simulink library "focLib"  (R2023a)
settings: Solver=VariableStepAuto  StartTime=0.0  StopTime=10.0  RelTol=1e-3
undefined symbols (not defined in the file): availableSpeedModes, ctrl_limits, Down, focp_tune_cur_Ki, focp_tune_cur_Kp, focp_tune_iq_max, focp_tune_iq_min, focp_tune_spd_Ki, focp_tune_spd_Kp, focp_tune_udc_max, GPTRIP1SEL, inverter_DRV8300, PI_params, pmsm_ECI6360, PU_System, target_f2838, Ts, Ts_motor, Ts_simulink, Ts_speed, TZ1, Up
libraries: simulink x31, c2802xlib x12, idelinklib_common x8, mcbcontrolslib x8, c280xlib x7, mcbpositiondecoderlib x7, slpidlib x5, c2837xDlib x2, c2838xlib x1, autolibpmsminterior x1, mcbplantlib x1, autolibpmsmexterior x1
(part 2 of 3)

== system focLib/Speed Control/Speed calculator ==
  Speed_Ref_PU : Inport
  speedMode : Inport  Port=2
  Gain : Gain  Gain=floor(PU_System.N_base/availableSpeedModes)  OutDataTypeStr=fixdt(1,32,17)  RndMeth=Ceiling
  Product : Product  OutDataTypeStr=fixdt(1,32,17)
  Subsystem : Subsystem  Commented=through
  rpm2PU : Gain  Gain=1/PU_System.N_base  OutMax=1  OutDataTypeStr=fixdt(1,32,17)
  N_Ref : Outport
  wires:
  Subsystem/1(Out1) -> N_Ref/1
  rpm2PU/1 -> Subsystem/1(In1)
  Product/1 -> rpm2PU/1
  speedMode/1 -> Product/1
  Gain/1 -> Product/2
  Speed_Ref_PU/1 -> Gain/1

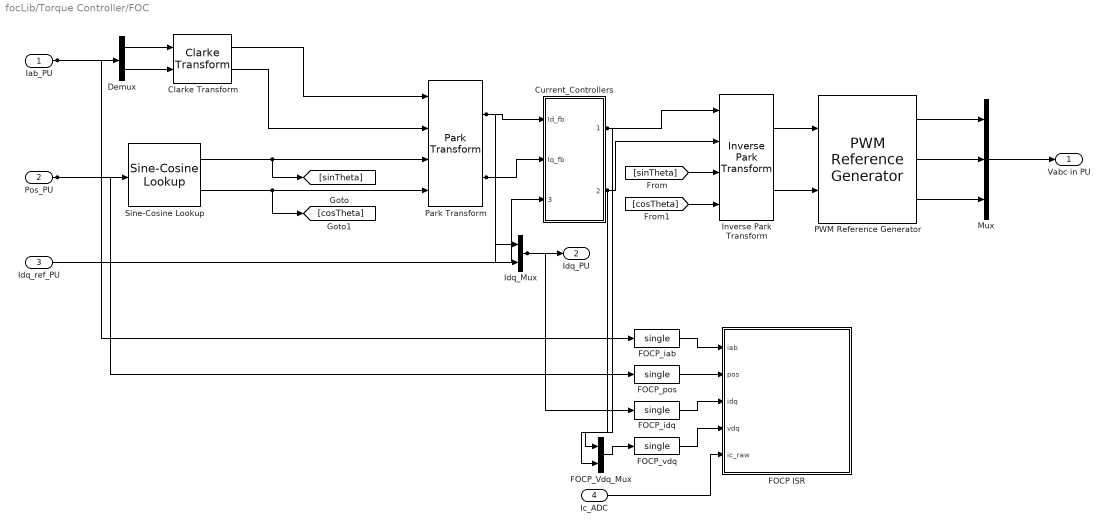
== system focLib/Torque Controller/FOC ==
  Iab_PU : Inport
  Pos_PU : Inport  Port=2
  Idq_ref_PU : Inport  Port=3
  Ic_ADC : Inport  Port=4
  Clarke Transform : mcbcontrolslib/Clarke Transform  VariantControl=Variant2
      settings: LibrarySourceBlock=mcbhdllib/Controls/Math Transforms/Clarke Transform
  Current_Controllers : Subsystem
  Demux : Demux  Outputs=2
  FOCP ISR : MATLAB Function  TreatAsAtomicUnit=on
  FOCP_Vdq_Mux : Mux  Inputs=2
  FOCP_iab : DataTypeConversion  OutDataTypeStr=single  SaturateOnIntegerOverflow=off  RndMeth=Floor
  FOCP_idq : DataTypeConversion  OutDataTypeStr=single  SaturateOnIntegerOverflow=off  RndMeth=Floor
  FOCP_pos : DataTypeConversion  OutDataTypeStr=single  SaturateOnIntegerOverflow=off  RndMeth=Floor
  FOCP_vdq : DataTypeConversion  OutDataTypeStr=single  SaturateOnIntegerOverflow=off  RndMeth=Floor
  Idq_Mux : Mux  Inputs=2
  Inverse Park Transform : mcbcontrolslib/Inverse Park Transform  AxisAlignment=D-axis
      settings: LibrarySourceBlock=mcbhdllib/Controls/Math Transforms/Inverse Park Transform
  Mux : Mux  Inputs=3
  PWM Reference Generator : mcbcontrolslib/PWM Reference Generator  inSignal=Valphabeta  modType=SVM: space vector modulation
      settings: LibrarySourceBlock=mcblib/Controls/Math Transforms/PWM Reference Generator
  Park Transform : mcbcontrolslib/Park Transform  AxisAlignment=D-axis
      settings: LibrarySourceBlock=mcbhdllib/Controls/Math Transforms/Park Transform
  Sine-Cosine Lookup : mcbcontrolslib/Sine-Cosine Lookup  AngleInput=Per-unit  N_points=1024
      settings: LibrarySourceBlock=mcblib/Controls/Math Transforms/Sine-Cosine Lookup
  Vabc in PU : Outport
  Idq_PU : Outport  Port=2
  wires:
  Current_Controllers/2(Vq_ref) -> Inverse Park Transform/2, FOCP_Vdq_Mux/2
  Current_Controllers/1(Vd_ref) -> Inverse Park Transform/1, FOCP_Vdq_Mux/1
  Pos_PU/1 -> Sine-Cosine Lookup/1, FOCP_pos/1
  Mux/1 -> Vabc in PU/1
  PWM Reference Generator/3 -> Mux/3
  PWM Reference Generator/2 -> Mux/2
  PWM Reference Generator/1 -> Mux/1
  Inverse Park Transform/2 -> PWM Reference Generator/2
  Inverse Park Transform/1 -> PWM Reference Generator/1
  [cosTheta] -> Inverse Park Transform/4
  [sinTheta] -> Inverse Park Transform/3
  Idq_ref_PU/1 -> Current_Controllers/3(Idq_ref_PU)
  Park Transform/2 -> Current_Controllers/2(Iq_fb), Idq_Mux/2
  Park Transform/1 -> Current_Controllers/1(Id_fb), Idq_Mux/1
  Sine-Cosine Lookup/2 -> Park Transform/4, [cosTheta]
  Sine-Cosine Lookup/1 -> Park Transform/3, [sinTheta]
  Clarke Transform/2 -> Park Transform/2
  Clarke Transform/1 -> Park Transform/1
  Demux/2 -> Clarke Transform/2
  Demux/1 -> Clarke Transform/1
  Iab_PU/1 -> Demux/1, FOCP_iab/1
  Idq_Mux/1 -> Idq_PU/1, FOCP_idq/1
  FOCP_iab/1 -> FOCP ISR/1(iab)
  FOCP_pos/1 -> FOCP ISR/2(pos)
  FOCP_idq/1 -> FOCP ISR/3(idq)
  FOCP_vdq/1 -> FOCP ISR/4(vdq)
  FOCP_Vdq_Mux/1 -> FOCP_vdq/1
  Ic_ADC/1 -> FOCP ISR/5(ic_raw)

== system focLib/Torque Controller/Iab_Meas_ADC ==
  ADC : c2802xlib/ADC  blkParamProc=C2000_Type4  ADCModule=B  samplingMode=Single sample mode  ADCResolution=12-bit (Single-ended input)  useSOC1=SOC0  useSOC2=SOC0_SOC1  SOCAcquisitionWindow=60  SOCTriggerSource=ePWM6_ADCSOCA  SOCInterruptTrigger=No ADCINT  Ts=-1  dType=uint16  postInterrupt=off  interruptSel=ADCINT1  ADCINTContinuous=on  endma=off  chdma=1  conv1=ADCINA0  conv2=ADCINA0 and ADCINB0  conv1_Type4=ADCIN0  conv2_Type4=ADCIN0 and ADCIN1
      settings: LibrarySourceBlock=c2838xlib/ADC
  ADC1 : c2802xlib/ADC  blkParamProc=C2000_Type4  ADCModule=B  samplingMode=Single sample mode  ADCResolution=12-bit (Single-ended input)  useSOC1=SOC1  useSOC2=SOC0_SOC1  SOCAcquisitionWindow=60  SOCTriggerSource=ePWM6_ADCSOCA  SOCInterruptTrigger=No ADCINT  Ts=-1  dType=uint16  postInterrupt=on  interruptSel=ADCINT1  ADCINTContinuous=on  endma=off  chdma=1  conv1=ADCINA0  conv2=ADCINA0 and ADCINB0  conv1_Type4=ADCIN2  conv2_Type4=ADCIN0 and ADCIN1
      settings: LibrarySourceBlock=c2838xlib/ADC
  ADC_IC : c2802xlib/ADC  blkParamProc=C2000_Type4  ADCModule=B  samplingMode=Single sample mode  ADCResolution=12-bit (Single-ended input)  useSOC1=SOC4  useSOC2=SOC0_SOC1  SOCAcquisitionWindow=60  SOCTriggerSource=ePWM6_ADCSOCA  SOCInterruptTrigger=No ADCINT  Ts=-1  dType=uint16  postInterrupt=off  interruptSel=ADCINT1  ADCINTContinuous=on  endma=off  chdma=1  conv1=ADCINA0  conv2=ADCINA0 and ADCINB0  conv1_Type4=ADCIN3  conv2_Type4=ADCIN0 and ADCIN1
      settings: LibrarySourceBlock=c2838xlib/ADC
  Mux : Mux  Inputs=2
  Iab_ADC : Outport
  Ic_ADC : Outport  Port=2
  wires:
  ADC1/1 -> Mux/2
  ADC/1 -> Mux/1
  Mux/1 -> Iab_ADC/1
  ADC_IC/1 -> Ic_ADC/1

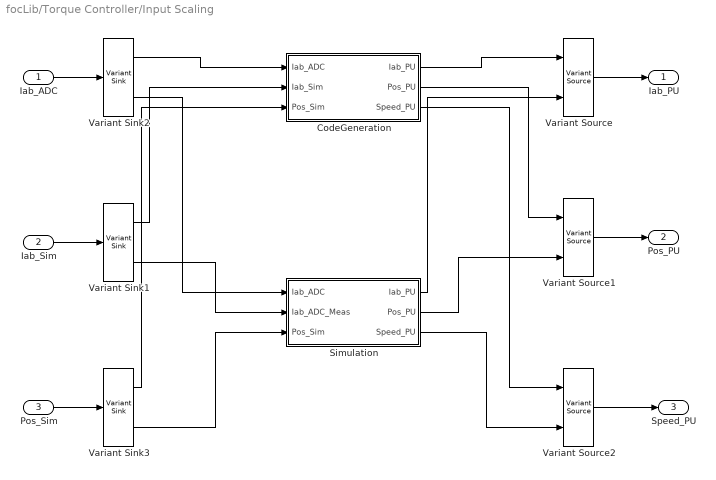
== system focLib/Torque Controller/Input Scaling ==
  Iab_ADC : Inport
  Iab_Sim : Inport  Port=2
  Pos_Sim : Inport  Port=3
  CodeGeneration : Subsystem
  Simulation : Subsystem
  Variant Sink1 : VariantSink  VariantControlMode=sim codegen switching
  Variant Sink2 : VariantSink  VariantControlMode=sim codegen switching
  Variant Sink3 : VariantSink  VariantControlMode=sim codegen switching
  Variant Source : VariantSource  VariantControlMode=sim codegen switching
  Variant Source1 : VariantSource  VariantControlMode=sim codegen switching
  Variant Source2 : VariantSource  VariantControlMode=sim codegen switching
  Iab_PU : Outport
  Pos_PU : Outport  Port=2
  Speed_PU : Outport  Port=3
  wires:
  Variant Source2/1 -> Speed_PU/1
  Variant Source1/1 -> Pos_PU/1
  Variant Source/1 -> Iab_PU/1
  CodeGeneration/3(Speed_PU) -> Variant Source2/1
  Simulation/3(Speed_PU) -> Variant Source2/2
  Simulation/2(Pos_PU) -> Variant Source1/2
  CodeGeneration/2(Pos_PU) -> Variant Source1/1
  Simulation/1(Iab_PU) -> Variant Source/2
  CodeGeneration/1(Iab_PU) -> Variant Source/1
  Variant Sink3/2 -> Simulation/3(Pos_Sim)
  Variant Sink1/2 -> Simulation/2(Iab_ADC_Meas)
  Variant Sink2/2 -> Simulation/1(Iab_ADC)
  Variant Sink3/1 -> CodeGeneration/3(Pos_Sim)
  Variant Sink1/1 -> CodeGeneration/2(Iab_Sim)
  Variant Sink2/1 -> CodeGeneration/1(Iab_ADC)
  Iab_ADC/1 -> Variant Sink2/1
  Iab_Sim/1 -> Variant Sink1/1
  Pos_Sim/1 -> Variant Sink3/1

== system focLib/Torque Controller/Output ==
  Scaled_DC : Inport
  CodeGeneration : Subsystem
  Scope : Scope
  Simulation : Subsystem
  Variant Sink : VariantSink  VariantControlMode=sim codegen switching
  Duty Cycle : Outport
  wires:
  Variant Sink/2 -> Simulation/1(Input)
  Variant Sink/1 -> CodeGeneration/1(In1)
  Simulation/1(Output) -> Duty Cycle/1, Scope/1
  Scaled_DC/1 -> Variant Sink/1

== system focLib/Torque Controller/PWM1 ==
  Scaled_DC_PWM1 : Inport
  Freemode_Sig : Inport  Port=2
  Constant : Constant  Value=0  OutDataTypeStr=fixdt(1,32,17)  SampleTime=-1
  Constant1 : Constant  OutDataTypeStr=fixdt(1,32,17)  SampleTime=-1
  Switch : Switch  Criteria=u2 > Threshold  SaturateOnIntegerOverflow=off  InputSameDT=off  OutDataTypeStr=Inherit: Same as first input
  Switch1 : Switch  Criteria=u2 > Threshold  SaturateOnIntegerOverflow=off  InputSameDT=off  OutDataTypeStr=Inherit: Same as first input
  WA : Outport
  WB : Outport  Port=2
  wires:
  Constant1/1 -> Switch1/1
  Constant/1 -> Switch/1
  Scaled_DC_PWM1/1 -> Switch1/3, Switch/3
  Switch1/1 -> WB/1
  Switch/1 -> WA/1
  Freemode_Sig/1 -> Switch/2, Switch1/2

== system focLib/Torque Controller/PWM2 ==
  Scaled_DC_PWM2 : Inport
  Freemode_Sig : Inport  Port=2
  Constant : Constant  Value=0  OutDataTypeStr=fixdt(1,32,17)  SampleTime=-1
  Constant1 : Constant  OutDataTypeStr=fixdt(1,32,17)  SampleTime=-1
  Switch : Switch  Criteria=u2 > Threshold  SaturateOnIntegerOverflow=off  InputSameDT=off  OutDataTypeStr=Inherit: Same as first input
  Switch1 : Switch  Criteria=u2 > Threshold  SaturateOnIntegerOverflow=off  InputSameDT=off  OutDataTypeStr=Inherit: Same as first input
  WA : Outport
  WB : Outport  Port=2
  wires:
  Scaled_DC_PWM2/1 -> Switch/3, Switch1/3
  Constant1/1 -> Switch1/1
  Freemode_Sig/1 -> Switch1/2, Switch/2
  Constant/1 -> Switch/1
  Switch1/1 -> WB/1
  Switch/1 -> WA/1

== system focLib/Torque Controller/PWM3 ==
  Scaled_DC_PWM3 : Inport
  Freemode_Sig : Inport  Port=2
  Constant : Constant  Value=0  OutDataTypeStr=fixdt(1,32,17)  SampleTime=-1
  Constant1 : Constant  OutDataTypeStr=fixdt(1,32,17)  SampleTime=-1
  Switch : Switch  Criteria=u2 > Threshold  SaturateOnIntegerOverflow=off  InputSameDT=off  OutDataTypeStr=Inherit: Same as first input
  Switch1 : Switch  Criteria=u2 > Threshold  SaturateOnIntegerOverflow=off  InputSameDT=off  OutDataTypeStr=Inherit: Same as first input
  WA : Outport
  WB : Outport  Port=2
  wires:
  Scaled_DC_PWM3/1 -> Switch/3, Switch1/3
  Constant1/1 -> Switch1/1
  Freemode_Sig/1 -> Switch/2, Switch1/2
  Constant/1 -> Switch/1
  Switch1/1 -> WB/1
  Switch/1 -> WA/1

== system focLib/Torque Controller/Scaling DutyCycles ==
  Unscaled_DC : Inport
  CodeGen : Subsystem
  Demux : Demux  Outputs=3
  Sim : Subsystem
  Variant Sink : VariantSink  VariantControlMode=sim codegen switching
  Variant Source : VariantSource  VariantControlMode=sim codegen switching
  Scaled_DC_PWM1 : Outport
  Scaled_DC_PWM2 : Outport  Port=2
  Scaled_DC_PWM3 : Outport  Port=3
  wires:
  CodeGen/1(Out1) -> Variant Source/1
  Variant Sink/1 -> CodeGen/1(In1)
  Variant Sink/2 -> Sim/1(In1)
  Sim/1(Out1) -> Variant Source/2
  Unscaled_DC/1 -> Variant Sink/1
  Variant Source/1 -> Demux/1
  Demux/3 -> Scaled_DC_PWM3/1
  Demux/2 -> Scaled_DC_PWM2/1
  Demux/1 -> Scaled_DC_PWM1/1

== system focLib/ADC Offset Function/Calculate ADC Offset /For Iterator Subsystem ==
  ADC_B_IN0 : c2802xlib/ADC  Priority=20  blkParamProc=C2000_Type4  ADCModule=B  samplingMode=Single sample mode  ADCResolution=12-bit (Single-ended input)  useSOC1=SOC2  useSOC2=SOC0_SOC1  SOCAcquisitionWindow=60  SOCTriggerSource=Software  SOCInterruptTrigger=No ADCINT  Ts=-1  dType=uint16  postInterrupt=off  interruptSel=ADCINT1  ADCINTContinuous=on  endma=off  chdma=1  conv1=ADCINA0  conv2=ADCINA0 and ADCINB0  conv1_Type4=ADCIN0  conv2_Type4=ADCIN0 and ADCIN1
  ADC_B_IN2 : c2802xlib/ADC  Priority=20  blkParamProc=C2000_Type4  ADCModule=B  samplingMode=Single sample mode  ADCResolution=12-bit (Single-ended input)  useSOC1=SOC3  useSOC2=SOC0_SOC1  SOCAcquisitionWindow=60  SOCTriggerSource=Software  SOCInterruptTrigger=No ADCINT  Ts=-1  dType=uint16  postInterrupt=off  interruptSel=ADCINT1  ADCINTContinuous=on  endma=off  chdma=1  conv1=ADCINA0  conv2=ADCINA0 and ADCINB0  conv1_Type4=ADCIN2  conv2_Type4=ADCIN0 and ADCIN1
  For Iterator : ForIterator  IterationLimit=16  IterationVariableDataType=uint16
  If : If  IfExpression=u1 > 8  ShowElse=off
  If Action Subsystem : Subsystem  TreatAsAtomicUnit=on
  Out1 : Outport
  Out2 : Outport  Port=2
  wires:
  If/1 -> If Action Subsystem/Action
  If Action Subsystem/2(Out2) -> Out2/1
  If Action Subsystem/1(Out1) -> Out1/1
  ADC_B_IN2/1 -> If Action Subsystem/2(In2)
  ADC_B_IN0/1 -> If Action Subsystem/1(In1)
  For Iterator/1 -> If/1

== system focLib/ADC Offset Function/Calculate ADC Offset /If Action Subsystem ==
  In1 : Inport
  Action Port : ActionPort
  Data Store Write1 : DataStoreWrite  DataStoreName=IaOffset  IndexOptions=Index vector (dialog)  Indices=1  OutputSizes=1
  wires:
  In1/1 -> Data Store Write1/1

== system focLib/ADC Offset Function/Calculate ADC Offset /If Action Subsystem1 ==
  Action Port : ActionPort
  Constant : Constant  Value=inverter_DRV8300.CtSensAOffset  OutDataTypeStr=Inherit: Inherit via back propagation
  Data Store Write1 : DataStoreWrite  DataStoreName=IaOffset  IndexOptions=Index vector (dialog)  Indices=1  OutputSizes=1
  wires:
  Constant/1 -> Data Store Write1/1

== system focLib/ADC Offset Function/Calculate ADC Offset /If Action Subsystem2 ==
  In1 : Inport
  Action Port : ActionPort
  Data Store Write2 : DataStoreWrite  DataStoreName=IbOffset  IndexOptions=Index vector (dialog)  Indices=1  OutputSizes=1
  wires:
  In1/1 -> Data Store Write2/1

== system focLib/ADC Offset Function/Calculate ADC Offset /If Action Subsystem3 ==
  Action Port : ActionPort
  Constant1 : Constant  Value=inverter_DRV8300.CtSensBOffset  OutDataTypeStr=Inherit: Inherit via back propagation
  Data Store Write2 : DataStoreWrite  DataStoreName=IbOffset  IndexOptions=Index vector (dialog)  Indices=1  OutputSizes=1
  wires:
  Constant1/1 -> Data Store Write2/1

== system focLib/Hall Sensor A/Capture Event Selection/Output 0 ==
  Action Port : ActionPort
  Constant : Constant  Value=0  OutDataTypeStr=boolean  SampleTime=-1
  Out1 : Outport
  wires:
  Constant/1 -> Out1/1

== system focLib/Hall Sensor A/Capture Event Selection/Output 1 ==
  Action Port : ActionPort
  Constant : Constant  OutDataTypeStr=boolean  SampleTime=-1
  Out1 : Outport
  wires:
  Constant/1 -> Out1/1

== system focLib/Hall Sensor B/Capture Event Selection/Output 0 ==
  Action Port : ActionPort
  Constant : Constant  Value=0  OutDataTypeStr=boolean  SampleTime=-1
  Out1 : Outport
  wires:
  Constant/1 -> Out1/1

== system focLib/Hall Sensor B/Capture Event Selection/Output 1 ==
  Action Port : ActionPort
  Constant : Constant  OutDataTypeStr=boolean  SampleTime=-1
  Out1 : Outport
  wires:
  Constant/1 -> Out1/1

== system focLib/Hall Sensor C/Capture Event Selection/Output 0 ==
  Action Port : ActionPort
  Constant : Constant  Value=0  OutDataTypeStr=boolean  SampleTime=-1
  Out1 : Outport
  wires:
  Constant/1 -> Out1/1

== system focLib/Hall Sensor C/Capture Event Selection/Output 1 ==
  Action Port : ActionPort
  Constant : Constant  OutDataTypeStr=boolean  SampleTime=-1
  Out1 : Outport
  wires:
  Constant/1 -> Out1/1

== system focLib/Input Controller/SpeedCommand_CodeGen/Check for SpeedRef ==
  In1 : Inport
  If : If  IfExpression=u1 > 4000
  If Action Subsystem : Subsystem  TreatAsAtomicUnit=on
  If Action Subsystem1 : Subsystem  TreatAsAtomicUnit=on
  Merge : Merge
  Out1 : Outport
  wires:
  If Action Subsystem1/1(Out1) -> Merge/2
  If Action Subsystem/1(Out1) -> Merge/1
  If/2 -> If Action Subsystem1/Action
  If/1 -> If Action Subsystem/Action
  Merge/1 -> Out1/1
  In1/1 -> If/1, If Action Subsystem1/1(In1)

== system focLib/Inverter and Motor - Plant Model/Simulation/Inverter ==
  Duty_abc : Inport
  Average-Value Inverter : mcbplantlib/Average-Value Inverter
  Constant2 : Constant  Value=inverter_DRV8300.V_dc  OutDataTypeStr=single  SampleTime=-1
  Data Type Conversion1 : DataTypeConversion  OutDataTypeStr=single  RndMeth=Simplest  SaturateOnIntegerOverflow=off
  Rate Transition3 : RateTransition  Integrity=off  OutPortSampleTime=Ts_inverter
  Vabc : Outport  VectorParamsAs1DForOutWhenUnconnected=off
  wires:
  Average-Value Inverter/1 -> Vabc/1
  Constant2/1 -> Average-Value Inverter/2
  Rate Transition3/1 -> Average-Value Inverter/1
  Data Type Conversion1/1 -> Rate Transition3/1
  Duty_abc/1 -> Data Type Conversion1/1

== system focLib/Inverter and Motor - Plant Model/Simulation/Load_Profile (Torque) ==
  Data Type Conversion : DataTypeConversion  OutDataTypeStr=single  SaturateOnIntegerOverflow=off  RndMeth=Floor
  IIR Filter : mcbcontrolslib/IIR Filter  VariantControl=Low Pass Filter  VariantSelect=Low-pass  Filter_constant=0.01  advancedSettings=off  Ts=50e-6  cutOff_freq=32.1525
  T_load : Step  Time=5  Before=0.1*pmsm_ECI6360.T_rated  After=0.1*pmsm_ECI6360.T_rated  SampleTime=Ts_simulink
  Load_Trq : Outport  VectorParamsAs1DForOutWhenUnconnected=off
  wires:
  IIR Filter/1 -> Load_Trq/1
  Data Type Conversion/1 -> IIR Filter/1
  T_load/1 -> Data Type Conversion/1

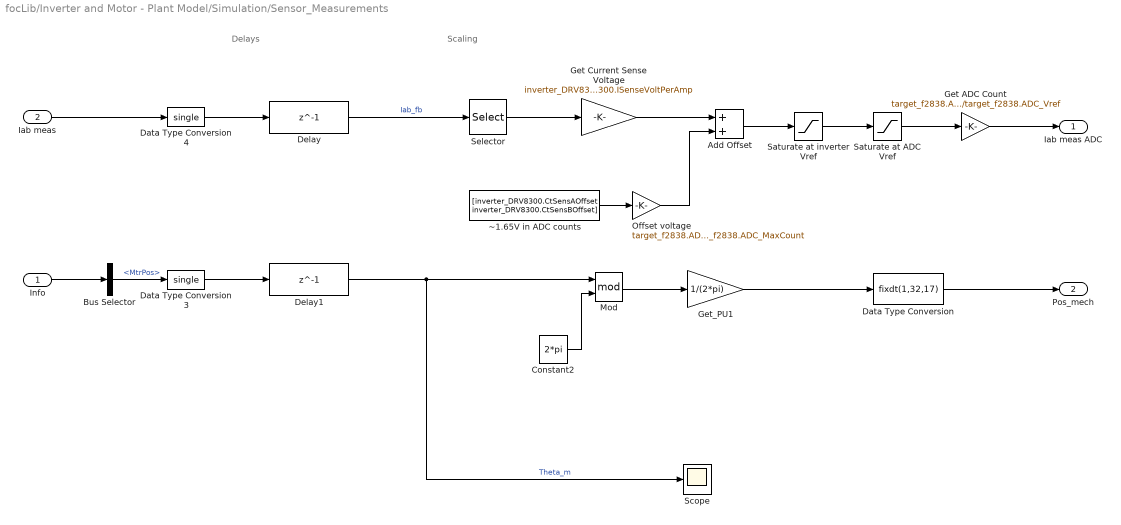
== system focLib/Inverter and Motor - Plant Model/Simulation/Sensor_Measurements ==
  note: Delays
  note: Scaling
  Info : Inport
  Iab meas : Inport  Port=2
  Add Offset : Sum  RndMeth=Simplest
  Bus Selector : BusSelector  OutputSignals=MtrPos
  Constant2 : Constant  Value=2*pi  OutDataTypeStr=single  SampleTime=-1
  Data Type Conversion : DataTypeConversion  OutDataTypeStr=fixdt(1,32,17)  SaturateOnIntegerOverflow=off  RndMeth=Floor
  Data Type Conversion3 : DataTypeConversion  OutDataTypeStr=single  RndMeth=Simplest  SaturateOnIntegerOverflow=off
  Data Type Conversion4 : DataTypeConversion  OutDataTypeStr=single  RndMeth=Simplest  SaturateOnIntegerOverflow=off
  Delay : Delay  DelayLength=1
  Delay1 : Delay  DelayLength=1
  Get ADC Count : Gain  Gain=target_f2838.ADC_MaxCount/target_f2838.ADC_Vref  OutMin=0  OutMax=target_f2838.ADC_MaxCount  OutDataTypeStr=uint16  RndMeth=Simplest
  Get Current Sense Voltage : Gain  Gain=inverter_DRV8300.invertingAmp*inverter_DRV8300.ISenseVoltPerAmp  RndMeth=Simplest  OutDataTypeStr=Inherit: Same as input
  Get_PU1 : Gain  Gain=1/(2*pi)  RndMeth=Simplest  OutDataTypeStr=Inherit: Same as input
  Mod : Math  Operator=mod
  Offset voltage : Gain  Gain=target_f2838.ADC_Vref / target_f2838.ADC_MaxCount  RndMeth=Simplest
  Saturate at ADC Vref : Saturate  UpperLimit=target_f2838.ADC_Vref  LowerLimit=0
  Saturate at inverter Vref : Saturate  UpperLimit=inverter_DRV8300.ISenseVref  LowerLimit=0
  Scope : Scope
  Selector : Selector  InputPortWidth=3  IndexOptions=Index vector (dialog)  Indices=[1 2]  OutputSizes=1
  ~1.65V in ADC counts : Constant  Value=[inverter_DRV8300.CtSensAOffset inverter_DRV8300.CtSensBOffset]  OutDataTypeStr=uint16  SampleTime=-1
  Iab meas ADC : Outport  VectorParamsAs1DForOutWhenUnconnected=off
  Pos_mech : Outport  Port=2
  wires:
  Data Type Conversion/1 -> Pos_mech/1
  Get Current Sense Voltage/1 -> Add Offset/1
  ~1.65V in ADC counts/1 -> Offset voltage/1
  Saturate at ADC Vref/1 -> Get ADC Count/1
  Offset voltage/1 -> Add Offset/2
  Get ADC Count/1 -> Iab meas ADC/1
  Add Offset/1 -> Saturate at inverter Vref/1
  Saturate at inverter Vref/1 -> Saturate at ADC Vref/1
  Selector/1 -> Get Current Sense Voltage/1
  Delay1/1 -> Mod/1, Scope/1  "Theta_m"
  Mod/1 -> Get_PU1/1
  Constant2/1 -> Mod/2
  Bus Selector/1 -> Data Type Conversion3/1  "<MtrPos>"
  Get_PU1/1 -> Data Type Conversion/1
  Data Type Conversion3/1 -> Delay1/1
  Info/1 -> Bus Selector/1
  Iab meas/1 -> Data Type Conversion4/1
  Data Type Conversion4/1 -> Delay/1
  Delay/1 -> Selector/1  "Iab_fb"

== system focLib/Speed Control/Mechanical_Freemode_Check/If Action Subsystem ==
  Action Port : ActionPort
  Constant : Constant  OutDataTypeStr=boolean  SampleTime=-1
  Out1 : Outport
  wires:
  Constant/1 -> Out1/1

== system focLib/Speed Control/Mechanical_Freemode_Check/If Action Subsystem1 ==
  Freemode_Sig_Dig : Inport
  Action Port : ActionPort
  Out1 : Outport
  wires:
  Freemode_Sig_Dig/1 -> Out1/1

== system focLib/Speed Control/Speed calculator/Subsystem ==
  In1 : Inport
  Data Type Conversion : DataTypeConversion  OutDataTypeStr=single  SaturateOnIntegerOverflow=off  RndMeth=Floor
  If : If  IfExpression=u1 > 0.94
  If Action Subsystem : Subsystem  TreatAsAtomicUnit=on
  If Action Subsystem1 : Subsystem  TreatAsAtomicUnit=on
  Merge : Merge
  Out1 : Outport
  wires:
  Data Type Conversion/1 -> If/1, If Action Subsystem1/1(In1)
  If Action Subsystem1/1(Out1) -> Merge/2
  If Action Subsystem/1(Out1) -> Merge/1
  Merge/1 -> Out1/1
  If/2 -> If Action Subsystem1/Action
  If/1 -> If Action Subsystem/Action
  In1/1 -> Data Type Conversion/1

== system focLib/Torque Controller/FOC/Current_Controllers ==
  Id_fb : Inport
  Iq_fb : Inport  Port=2
  Idq_ref_PU : Inport  Port=3
  DQ Limiter : mcbcontrolslib/DQ Limiter  satMethodInputType=Specify via dialog  satMethodSelected=D-Q equivalence  satLimitInputType=Specify via dialog  Vmax=0.95
  Demux : Demux  Outputs=2
  PI_Controller_Id : Subsystem
  PI_Controller_Iq : Subsystem
  Sum : Sum  Inputs=|+-
  Sum1 : Sum  Inputs=|+-
  Terminator : Terminator
  Vd_ref : Outport  VectorParamsAs1DForOutWhenUnconnected=off
  Vq_ref : Outport  Port=2  VectorParamsAs1DForOutWhenUnconnected=off
  wires:
  PI_Controller_Iq/1(V_ref) -> DQ Limiter/2
  PI_Controller_Id/1(V_ref) -> DQ Limiter/1
  Sum1/1 -> PI_Controller_Iq/1(Iq_in)
  Id_fb/1 -> Sum/2
  Sum/1 -> PI_Controller_Id/1(Id_in)
  DQ Limiter/3 -> Terminator/1
  DQ Limiter/2 -> Vq_ref/1
  DQ Limiter/1 -> Vd_ref/1
  Demux/2 -> Sum1/1  "Iq_Ref"
  Demux/1 -> Sum/1  "Id_Ref"
  Idq_ref_PU/1 -> Demux/1
  Iq_fb/1 -> Sum1/2

== system focLib/Torque Controller/Input Scaling/CodeGeneration ==
  Iab_ADC : Inport
  Iab_Sim : Inport  Port=2
  Pos_Sim : Inport  Port=3
  Calculate Position from Hall : Subsystem  TreatAsAtomicUnit=on
  Convert ADC value to PU : Subsystem
  Terminator : Terminator
  Terminator1 : Terminator
  Iab_PU : Outport
  Pos_PU : Outport  Port=2
  Speed_PU : Outport  Port=3
  wires:
  Calculate Position from Hall/2(Speed_PU) -> Speed_PU/1
  Pos_Sim/1 -> Terminator1/1
  Iab_Sim/1 -> Terminator/1
  Calculate Position from Hall/1(Pos_PU) -> Pos_PU/1
  Iab_ADC/1 -> Convert ADC value to PU/1(Iab_ADC)
  Convert ADC value to PU/1(Iab_PU) -> Iab_PU/1

== system focLib/Torque Controller/Input Scaling/Simulation ==
  Iab_ADC : Inport
  Iab_ADC_Meas : Inport  Port=2
  Pos_Sim : Inport  Port=3
  Convert Iab to PU : Subsystem
  Convert Pos to PU : Subsystem
  Terminator : Terminator
  Iab_PU : Outport
  Pos_PU : Outport  Port=2
  Speed_PU : Outport  Port=3
  wires:
  Iab_ADC_Meas/1 -> Convert Iab to PU/1(Iab_ADC_Sim)
  Convert Iab to PU/1(Iab_PU) -> Iab_PU/1
  Pos_Sim/1 -> Convert Pos to PU/1(Pos_Sim)
  Convert Pos to PU/2(Speed_PU) -> Speed_PU/1
  Convert Pos to PU/1(Theta) -> Pos_PU/1
  Iab_ADC/1 -> Terminator/1

== system focLib/Torque Controller/Output/CodeGeneration ==
  In1 : Inport
  CMPSS3_COMPH : c2837xDlib/CMPSS  Module=CMPSS3_COMPH  NegativeInput=Internal DAC  DacValueSourceSel=DAC module  DacValueVia=Dialog  DACHValue=ctrl_limits.cmpss_dac_hi  DACLValue=0  DACInitValue=0  RampMaxRefVal=0  RampInitRefVal=0  RampDecVal=0  RampInitDecVal=0  RampDelayVal=0  RampInitDelayVal=0  EnableLatchOut=off  EnableLatchClear=off  SampleTime=-1
      settings: LibrarySourceBlock=c2838xlib/CMPSS
  CMPSS3_COMPH_Term1 : Terminator
  CMPSS3_COMPL : c2837xDlib/CMPSS  Module=CMPSS3_COMPL  NegativeInput=Internal DAC  DacValueSourceSel=DAC module  DacValueVia=Dialog  DACHValue=0  DACLValue=ctrl_limits.cmpss_dac_lo  DACInitValue=0  RampMaxRefVal=0  RampInitRefVal=0  RampDecVal=0  RampInitDecVal=0  RampDelayVal=0  RampInitDelayVal=0  EnableLatchOut=off  EnableLatchClear=off  SampleTime=-1
      settings: LibrarySourceBlock=c2838xlib/CMPSS
  CMPSS3_COMPL_Term1 : Terminator
  Demux : Demux  Outputs=6
  Gain : Gain  Gain=target_f2838.PWM_Counter_Period  OutDataTypeStr=fixdt(1,32,17)
  ePWM1 : c2802xlib/ePWM  PwmType=C2000_Type4_F2838x  useModule=ePWM6  ePWMxLINKTBPRD=Not Linked  periodUnits=Clock cycles  timerSource=Specify via dialog  timerPeriod_clk=target_f2838.PWM_Counter_Period  timerPeriod_sec=0.0001  tbshadow=Counter equals to zero  countingMode=Up-Down  phaseActiveEnable=Disable  phaseDirection=Count down after sync  phaseActive=0  synchronizationEnable=off  dcaevt1Sync=off  dcbevt1Sync=off  synchronizationOption=Disable  dcbevt1SyncOut=off  dcaevt1SyncOut=off  cmpdSyncOut=off  cmpcSyncOut=off  cmpbSyncOut=off  zeroSyncOut=on  swfSyncOut=off  perSynchronizationOption=Counter equals to period (CTR=PRD)  clockPrescale=1  HSclockPrescale=1  enswap=off  ePWMxAStatus=on  ePWMxAactionLogic1=Do nothing  ePWMxAactionLogic2=Do nothing  ePWMxAactionLogic3=Clear  ePWMxAactionLogic4=Set  ePWMxAactionLogic5=Do nothing  ePWMxAactionLogic6=Do nothing  ePWMxACSFenable=off  ePWMxACSFvalue=Forcing disable  ePWMxASFreload=Zero  ePWMxBStatus=on  ePWMxBactionLogic1=Do nothing  ePWMxBactionLogic2=Do nothing  ePWMxBactionLogic3=Do nothing  ePWMxBactionLogic4=Do nothing  ePWMxBactionLogic5=Clear  ePWMxBactionLogic6=Set  ePWMxBCSFenable=off  ePWMxBCSFvalue=Forcing disable  ePWMxBSFreload=Zero  ePWNxBOutWay=off  ePWMxLINKCMPA=Not Linked  CMPAUnits=Clock cycles  CMPASource=Input port  CMPAValue_per=50  CMPAValue_clk=floor(target_f2838.PWM_Counter_Period/2)  enCMPAshadow=Counter equals to zero (CTR=Zero)  ePWMxLINKCMPB=Not Linked  CMPBUnits=Clock cycles  CMPBSource=Input port  CMPBValue_per=50  CMPBValue_clk=floor(target_f2838.PWM_Counter_Period/2)  enCMPBshadow=Counter equals to zero (CTR=Zero)  ePWMxLINKCMPC=Not Linked  CMPCUnits=Clock cycles  CMPCSource=Specify via dialog  CMPCValue_per=50  CMPCValue_clk=32000  enCMPCshadow=Counter equals to zero (CTR=Zero)  ePWMxLINKCMPD=Not Linked  CMPDUnits=Clock cycles  CMPDSource=Specify via dialog  CMPDValue_per=50  CMPDValue_clk=32000  enCMPDshadow=Counter equals to zero (CTR=Zero)  enableDBePWMxA=off  enableDBePWMxB=off  enhalfcycle=off  DBpolarity=Active high complementary (AHC)  DBedgeDelay=Positive  DBSource_ePWMxA=ePWMxA  DBSource_ePWMxB=ePWMxA  DBPeriodUnits=Clock cycles  DBperiodSource=Specify via dialog  REDperiod=15  FEDperiod=15  REDperiod_sec=0  FEDperiod_sec=0  LoadModeDBRED=Immediate without using shadow  LoadModeDBFED=Immediate without using shadow  adcstartModuleA=on  adcrequestEventA=First event  adcstartEventA=Digital Compare Module A Event 1 start of conversion (DCAEVT1.soc)  adcstartEventA_type2=Counter equals to period (CTR=PRD)  adcstartModuleB=off  adcrequestEventB=First event  adcstartEventB=Counter equals to zero (CTR=Zero)  adcstartEventB_type2=Counter equals to zero (CTR=Zero)  intEn=off  intPrd=First event  intSel=Counter equals to zero (CTR=Zero)  intSel_type2=Counter equals to zero (CTR=Zero)  hrpe=off  enHRPWM=off  HRPWM_LoadMode=Counter equals to period (CTR=PRD)  HRPWM_CTLMode=Duty or Period control mode  HRPWM_EDGMode=Both edge  hrpeb=off  enHRPWMB=off  HRPWM_LoadModeB=Counter equals to zero (CTR=ZERO)  HRPWM_CTLModeB=Duty or Period control mode  HRPWM_EDGModeB=Both edge  enHRDBRED=off  enHRDBFED=off  enSFO=on  enautoconv=on  chopperEnable=off  chopperFrequency=1  chopperFirstwidth=1  chopperDuty=12.5%  tripZonesource=Specify via dialog  tzselOSHT1=off  tzselOSHT2=off  tzselOSHT3=off  tzselOSHDCAEV1=on  tzselOSHDCBEV1=off  tzselCBC1=off  tzselCBC2=off  tzselCBC3=off  tzselCBCDCAEV2=off  tzselCBCDCBEV2=off  tzselOSHT4=off  tzselOSHT5=off  tzselOSHT6=off  tzselCBC4=off  tzselCBC5=off  tzselCBC6=off  enTzOstIntr=off  enTzCbcIntr=off  enTzDCAEVT1Intr=off  enTzDCAEVT2Intr=off  enTzDCBEVT1Intr=off  enTzDCBEVT2Intr=off  ePWMxAforced=Low  ePWMxBforced=High  DCAEVT1forced=No action  DCBEVT1forced=No action  DCAEVT2forced=No action  DCBEVT2forced=No action  dcah=Trip Zone 1 input (TZ1)  dcal=Trip Zone 2 input (TZ2)  dcbh=Trip Zone 1 input (TZ1)  dcbl=Trip Zone 2 input (TZ2)  dcah_type2=GPTRIP4SEL  dcal_type2=GPTRIP1SEL/(TZ1)  dcbh_type2=GPTRIP1SEL/(TZ1)  dcbl_type2=GPTRIP1SEL/(TZ1)  gendcaevt1=DCAH=high and DCAL=don't care  gendcaevt2=Event disabled  gendcbevt1=Event disabled  gendcbevt2=Event disabled  dcaevt1src=DCAEVT1 with async  dcaevt2src=DCAEVT2 with sync  dcbevt1src=DCBEVT1 with sync  dcbevt2src=DCBEVT2 with sync  pulsesel=Counter equals to zero (CTR=Zero)  blankinv=off  blankoffset=0  blankwidth=0  evsrcsel=Filtered version of DCAEVT1 (DCAEVT1FILT)  encape=off
      settings: LibrarySourceBlock=c2838xlib/ePWM
  ePWM2 : c2802xlib/ePWM  PwmType=C2000_Type4_F2838x  useModule=ePWM7  ePWMxLINKTBPRD=Not Linked  periodUnits=Clock cycles  timerSource=Specify via dialog  timerPeriod_clk=target_f2838.PWM_Counter_Period  timerPeriod_sec=0.0001  tbshadow=Counter equals to zero  countingMode=Up-Down  phaseActiveEnable=Set counter to phase value specified via dialog  phaseDirection=Count up after sync  phaseActive=0  synchronizationEnable=off  dcaevt1Sync=off  dcbevt1Sync=off  synchronizationOption=Disable  dcbevt1SyncOut=off  dcaevt1SyncOut=off  cmpdSyncOut=off  cmpcSyncOut=off  cmpbSyncOut=off  zeroSyncOut=off  swfSyncOut=on  perSynchronizationOption=Counter equals to period (CTR=PRD)  clockPrescale=1  HSclockPrescale=1  enswap=off  ePWMxAStatus=on  ePWMxAactionLogic1=Do nothing  ePWMxAactionLogic2=Do nothing  ePWMxAactionLogic3=Clear  ePWMxAactionLogic4=Set  ePWMxAactionLogic5=Do nothing  ePWMxAactionLogic6=Do nothing  ePWMxACSFenable=off  ePWMxACSFvalue=Forcing disable  ePWMxASFreload=Zero  ePWMxBStatus=on  ePWMxBactionLogic1=Do nothing  ePWMxBactionLogic2=Do nothing  ePWMxBactionLogic3=Do nothing  ePWMxBactionLogic4=Do nothing  ePWMxBactionLogic5=Clear  ePWMxBactionLogic6=Set  ePWMxBCSFenable=off  ePWMxBCSFvalue=Forcing disable  ePWMxBSFreload=Zero  ePWNxBOutWay=off  ePWMxLINKCMPA=Not Linked  CMPAUnits=Clock cycles  CMPASource=Input port  CMPAValue_per=50  CMPAValue_clk=floor(target_f2838.PWM_Counter_Period/2)  enCMPAshadow=Counter equals to zero (CTR=Zero)  ePWMxLINKCMPB=Not Linked  CMPBUnits=Clock cycles  CMPBSource=Input port  CMPBValue_per=50  CMPBValue_clk=floor(target_f2838.PWM_Counter_Period/2)  enCMPBshadow=Counter equals to zero (CTR=Zero)  ePWMxLINKCMPC=Not Linked  CMPCUnits=Clock cycles  CMPCSource=Specify via dialog  CMPCValue_per=50  CMPCValue_clk=32000  enCMPCshadow=Counter equals to zero (CTR=Zero)  ePWMxLINKCMPD=Not Linked  CMPDUnits=Clock cycles  CMPDSource=Specify via dialog  CMPDValue_per=50  CMPDValue_clk=32000  enCMPDshadow=Counter equals to zero (CTR=Zero)  enableDBePWMxA=off  enableDBePWMxB=off  enhalfcycle=off  DBpolarity=Active high complementary (AHC)  DBedgeDelay=Positive  DBSource_ePWMxA=ePWMxA  DBSource_ePWMxB=ePWMxA  DBPeriodUnits=Clock cycles  DBperiodSource=Specify via dialog  REDperiod=15  FEDperiod=15  REDperiod_sec=0  FEDperiod_sec=0  LoadModeDBRED=Immediate without using shadow  LoadModeDBFED=Immediate without using shadow  adcstartModuleA=off  adcrequestEventA=First event  adcstartEventA=Digital Compare Module A Event 1 start of conversion (DCAEVT1.soc)  adcstartEventA_type2=Counter equals to zero (CTR=Zero)  adcstartModuleB=off  adcrequestEventB=First event  adcstartEventB=Counter equals to zero (CTR=Zero)  adcstartEventB_type2=Counter equals to zero (CTR=Zero)  intEn=off  intPrd=First event  intSel=Counter equals to zero (CTR=Zero)  intSel_type2=Counter equals to zero (CTR=Zero)  hrpe=off  enHRPWM=off  HRPWM_LoadMode=Counter equals to period (CTR=PRD)  HRPWM_CTLMode=Duty or Period control mode  HRPWM_EDGMode=Both edge  hrpeb=off  enHRPWMB=off  HRPWM_LoadModeB=Counter equals to zero (CTR=ZERO)  HRPWM_CTLModeB=Duty or Period control mode  HRPWM_EDGModeB=Both edge  enHRDBRED=off  enHRDBFED=off  enSFO=on  enautoconv=on  chopperEnable=off  chopperFrequency=1  chopperFirstwidth=1  chopperDuty=12.5%  tripZonesource=Specify via dialog  tzselOSHT1=off  tzselOSHT2=off  tzselOSHT3=off  tzselOSHDCAEV1=on  tzselOSHDCBEV1=off  tzselCBC1=off  tzselCBC2=off  tzselCBC3=off  tzselCBCDCAEV2=off  tzselCBCDCBEV2=off  tzselOSHT4=off  tzselOSHT5=off  tzselOSHT6=off  tzselCBC4=off  tzselCBC5=off  tzselCBC6=off  enTzOstIntr=off  enTzCbcIntr=off  enTzDCAEVT1Intr=off  enTzDCAEVT2Intr=off  enTzDCBEVT1Intr=off  enTzDCBEVT2Intr=off  ePWMxAforced=Low  ePWMxBforced=High  DCAEVT1forced=No action  DCBEVT1forced=No action  DCAEVT2forced=No action  DCBEVT2forced=No action  dcah=Trip Zone 1 input (TZ1)  dcal=Trip Zone 2 input (TZ2)  dcbh=Trip Zone 1 input (TZ1)  dcbl=Trip Zone 2 input (TZ2)  dcah_type2=GPTRIP4SEL  dcal_type2=GPTRIP1SEL/(TZ1)  dcbh_type2=GPTRIP1SEL/(TZ1)  dcbl_type2=GPTRIP1SEL/(TZ1)  gendcaevt1=DCAH=high and DCAL=don't care  gendcaevt2=Event disabled  gendcbevt1=Event disabled  gendcbevt2=Event disabled  dcaevt1src=DCAEVT1 with async  dcaevt2src=DCAEVT2 with sync  dcbevt1src=DCBEVT1 with sync  dcbevt2src=DCBEVT2 with sync  pulsesel=Counter equals to zero (CTR=Zero)  blankinv=off  blankoffset=0  blankwidth=0  evsrcsel=Filtered version of DCAEVT1 (DCAEVT1FILT)  encape=off
      settings: LibrarySourceBlock=c2838xlib/ePWM
  ePWM3 : c2802xlib/ePWM  PwmType=C2000_Type4_F2838x  useModule=ePWM8  ePWMxLINKTBPRD=Not Linked  periodUnits=Clock cycles  timerSource=Specify via dialog  timerPeriod_clk=target_f2838.PWM_Counter_Period  timerPeriod_sec=0.0001  tbshadow=Counter equals to zero  countingMode=Up-Down  phaseActiveEnable=Set counter to phase value specified via dialog  phaseDirection=Count up after sync  phaseActive=0  synchronizationEnable=off  dcaevt1Sync=off  dcbevt1Sync=off  synchronizationOption=Disable  dcbevt1SyncOut=off  dcaevt1SyncOut=off  cmpdSyncOut=off  cmpcSyncOut=off  cmpbSyncOut=off  zeroSyncOut=off  swfSyncOut=on  perSynchronizationOption=Counter equals to period (CTR=PRD)  clockPrescale=1  HSclockPrescale=1  enswap=off  ePWMxAStatus=on  ePWMxAactionLogic1=Do nothing  ePWMxAactionLogic2=Do nothing  ePWMxAactionLogic3=Clear  ePWMxAactionLogic4=Set  ePWMxAactionLogic5=Do nothing  ePWMxAactionLogic6=Do nothing  ePWMxACSFenable=off  ePWMxACSFvalue=Forcing disable  ePWMxASFreload=Zero  ePWMxBStatus=on  ePWMxBactionLogic1=Do nothing  ePWMxBactionLogic2=Do nothing  ePWMxBactionLogic3=Do nothing  ePWMxBactionLogic4=Do nothing  ePWMxBactionLogic5=Clear  ePWMxBactionLogic6=Set  ePWMxBCSFenable=off  ePWMxBCSFvalue=Forcing disable  ePWMxBSFreload=Zero  ePWNxBOutWay=off  ePWMxLINKCMPA=Not Linked  CMPAUnits=Clock cycles  CMPASource=Input port  CMPAValue_per=50  CMPAValue_clk=floor(target_f2838.PWM_Counter_Period/2)  enCMPAshadow=Counter equals to zero (CTR=Zero)  ePWMxLINKCMPB=Not Linked  CMPBUnits=Clock cycles  CMPBSource=Input port  CMPBValue_per=50  CMPBValue_clk=floor(target_f2838.PWM_Counter_Period/2)  enCMPBshadow=Counter equals to zero (CTR=Zero)  ePWMxLINKCMPC=Not Linked  CMPCUnits=Clock cycles  CMPCSource=Specify via dialog  CMPCValue_per=50  CMPCValue_clk=32000  enCMPCshadow=Counter equals to zero (CTR=Zero)  ePWMxLINKCMPD=Not Linked  CMPDUnits=Clock cycles  CMPDSource=Specify via dialog  CMPDValue_per=50  CMPDValue_clk=32000  enCMPDshadow=Counter equals to zero (CTR=Zero)  enableDBePWMxA=off  enableDBePWMxB=off  enhalfcycle=off  DBpolarity=Active high complementary (AHC)  DBedgeDelay=Positive  DBSource_ePWMxA=ePWMxA  DBSource_ePWMxB=ePWMxA  DBPeriodUnits=Clock cycles  DBperiodSource=Specify via dialog  REDperiod=15  FEDperiod=15  REDperiod_sec=0  FEDperiod_sec=0  LoadModeDBRED=Immediate without using shadow  LoadModeDBFED=Immediate without using shadow  adcstartModuleA=off  adcrequestEventA=First event  adcstartEventA=Digital Compare Module A Event 1 start of conversion (DCAEVT1.soc)  adcstartEventA_type2=Counter equals to zero (CTR=Zero)  adcstartModuleB=off  adcrequestEventB=First event  adcstartEventB=Counter equals to zero (CTR=Zero)  adcstartEventB_type2=Counter equals to zero (CTR=Zero)  intEn=off  intPrd=First event  intSel=Counter equals to zero (CTR=Zero)  intSel_type2=Counter equals to zero (CTR=Zero)  hrpe=off  enHRPWM=off  HRPWM_LoadMode=Counter equals to period (CTR=PRD)  HRPWM_CTLMode=Duty or Period control mode  HRPWM_EDGMode=Both edge  hrpeb=off  enHRPWMB=off  HRPWM_LoadModeB=Counter equals to zero (CTR=ZERO)  HRPWM_CTLModeB=Duty or Period control mode  HRPWM_EDGModeB=Both edge  enHRDBRED=off  enHRDBFED=off  enSFO=on  enautoconv=on  chopperEnable=off  chopperFrequency=1  chopperFirstwidth=1  chopperDuty=12.5%  tripZonesource=Specify via dialog  tzselOSHT1=off  tzselOSHT2=off  tzselOSHT3=off  tzselOSHDCAEV1=on  tzselOSHDCBEV1=off  tzselCBC1=off  tzselCBC2=off  tzselCBC3=off  tzselCBCDCAEV2=off  tzselCBCDCBEV2=off  tzselOSHT4=off  tzselOSHT5=off  tzselOSHT6=off  tzselCBC4=off  tzselCBC5=off  tzselCBC6=off  enTzOstIntr=off  enTzCbcIntr=off  enTzDCAEVT1Intr=off  enTzDCAEVT2Intr=off  enTzDCBEVT1Intr=off  enTzDCBEVT2Intr=off  ePWMxAforced=Low  ePWMxBforced=High  DCAEVT1forced=No action  DCBEVT1forced=No action  DCAEVT2forced=No action  DCBEVT2forced=No action  dcah=Trip Zone 1 input (TZ1)  dcal=Trip Zone 2 input (TZ2)  dcbh=Trip Zone 1 input (TZ1)  dcbl=Trip Zone 2 input (TZ2)  dcah_type2=GPTRIP4SEL  dcal_type2=GPTRIP1SEL/(TZ1)  dcbh_type2=GPTRIP1SEL/(TZ1)  dcbl_type2=GPTRIP1SEL/(TZ1)  gendcaevt1=DCAH=high and DCAL=don't care  gendcaevt2=Event disabled  gendcbevt1=Event disabled  gendcbevt2=Event disabled  dcaevt1src=DCAEVT1 with async  dcaevt2src=DCAEVT2 with sync  dcbevt1src=DCBEVT1 with sync  dcbevt2src=DCBEVT2 with sync  pulsesel=Counter equals to zero (CTR=Zero)  blankinv=off  blankoffset=0  blankwidth=0  evsrcsel=Filtered version of DCAEVT1 (DCAEVT1FILT)  encape=off
      settings: LibrarySourceBlock=c2838xlib/ePWM
  wires:
  Gain/1 -> Demux/1
  Demux/3 -> ePWM2/1
  Demux/4 -> ePWM2/2
  Demux/5 -> ePWM3/1
  Demux/2 -> ePWM1/2
  Demux/6 -> ePWM3/2
  Demux/1 -> ePWM1/1
  In1/1 -> Gain/1
  CMPSS3_COMPH/1 -> CMPSS3_COMPH_Term1/1
  CMPSS3_COMPL/1 -> CMPSS3_COMPL_Term1/1

== system focLib/Torque Controller/Output/Simulation ==
  Input : Inport
  Demux : Demux  Outputs=6
  Mux : Mux  Inputs=3
  Terminator : Terminator
  Terminator1 : Terminator
  Terminator2 : Terminator
  Output : Outport
  wires:
  Mux/1 -> Output/1
  Input/1 -> Demux/1
  Demux/3 -> Mux/2
  Demux/2 -> Terminator2/1
  Demux/6 -> Terminator/1
  Demux/1 -> Mux/1
  Demux/4 -> Terminator1/1
  Demux/5 -> Mux/3

== system focLib/Torque Controller/Scaling DutyCycles/CodeGen ==
  In1 : Inport
  Constant : Constant  Value=0.5  OutDataTypeStr=fixdt(1,32,17)  SampleTime=-1
  Gain : Gain  Gain=-0.5  RndMeth=Simplest  OutDataTypeStr=Inherit: Same as input
  Sum : Sum  Inputs=|++
  Out1 : Outport
  wires:
  Gain/1 -> Sum/1
  Constant/1 -> Sum/2
  Sum/1 -> Out1/1
  In1/1 -> Gain/1

== system focLib/Torque Controller/Scaling DutyCycles/Sim ==
  In1 : Inport
  Constant : Constant  Value=0.5  OutDataTypeStr=fixdt(1,32,17)  SampleTime=-1
  Gain : Gain  Gain=-0.5  RndMeth=Simplest  OutDataTypeStr=Inherit: Same as input
  Sum : Sum  Inputs=|++
  Out1 : Outport
  wires:
  Gain/1 -> Sum/1
  Constant/1 -> Sum/2
  Sum/1 -> Out1/1
  In1/1 -> Gain/1

== system focLib/ADC Offset Function/Calculate ADC Offset /For Iterator Subsystem/If Action Subsystem ==
  In1 : Inport
  In2 : Inport  Port=2
  Action Port : ActionPort
  Memory : Memory  InheritSampleTime=on
  Memory1 : Memory  InheritSampleTime=on
  Sum : Sum
  Sum1 : Sum
  Out1 : Outport
  Out2 : Outport  Port=2
  wires:
  Memory1/1 -> Sum1/2
  Sum1/1 -> Memory1/1, Out2/1
  Memory/1 -> Sum/2
  In2/1 -> Sum1/1
  Sum/1 -> Memory/1, Out1/1
  In1/1 -> Sum/1

== system focLib/Input Controller/SpeedCommand_CodeGen/Check for SpeedRef/If Action Subsystem ==
  Action Port : ActionPort
  Constant : Constant  Value=4095  OutDataTypeStr=uint16  SampleTime=-1
  Out1 : Outport
  wires:
  Constant/1 -> Out1/1

== system focLib/Input Controller/SpeedCommand_CodeGen/Check for SpeedRef/If Action Subsystem1 ==
  In1 : Inport
  Action Port : ActionPort
  Out1 : Outport
  wires:
  In1/1 -> Out1/1

== system focLib/Speed Control/Speed calculator/Subsystem/If Action Subsystem ==
  Action Port : ActionPort
  Constant : Constant  OutDataTypeStr=fixdt(1,32,17)  SampleTime=-1
  Out1 : Outport
  wires:
  Constant/1 -> Out1/1

== system focLib/Speed Control/Speed calculator/Subsystem/If Action Subsystem1 ==
  In1 : Inport
  Action Port : ActionPort
  Data Type Conversion : DataTypeConversion  OutDataTypeStr=fixdt(1,32,17)  SaturateOnIntegerOverflow=off  RndMeth=Floor
  Out1 : Outport
  wires:
  Data Type Conversion/1 -> Out1/1
  In1/1 -> Data Type Conversion/1

== system focLib/Torque Controller/FOC/Current_Controllers/PI_Controller_Id ==
  Id_in : Inport
  Data Store Read1 : DataStoreRead  Commented=on  DataStoreName=Enable  IndexOptions=Index vector (dialog)  Indices=1  OutputSizes=1
  Discrete PI Controller with anti-windup & reset : slpidlib/PID Controller  Commented=on  Controller=PI  Form=Parallel  TimeDomain=Discrete-time  UseExternalTs=off  SampleTime=-1  IntegratorMethod=Forward Euler  FilterMethod=Forward Euler  ControllerParametersSource=external  P=1  I=1  UseKiTs=on  D=0  N=100  UseFilter=on  TunerSelectOption=Transfer Function Based (PID Tuner App)  InitialConditionSource=external  InitialConditionForIntegrator=0  InitialConditionForFilter=0  DifferentiatorICPrevScaledInput=0  ExternalReset=level  TrackingMode=off  Kt=1  LimitOutput=on  SatLimitsSource=internal  UpperSaturationLimit=1  LowerSaturationLimit=-1  LinearizeAsGain=on  AntiWindupMode=clamping  Kb=1  LimitIntegrator=off  UpperIntegratorSaturationLimit=inf  LowerIntegratorSaturationLimit=-inf  RndMeth=Simplest  PGainOutDataTypeStr=single  PProdOutDataTypeStr=single  POutMin=[]  POutMax=[]  IGainOutDataTypeStr=single  IProdOutDataTypeStr=single  IOutMin=[]  IOutMax=[]  DOutMin=[]  DOutMax=[]  NOutMin=[]  NOutMax=[]  SumOutDataTypeStr=single  SumOutMin=[]  SumOutMax=[]  SaturationOutDataTypeStr=single  SaturationOutMin=[]  SaturationOutMax=[]  PParamMin=[]  PParamMax=[]  IParamMin=[]  IParamMax=[]  DParamMin=[]  DParamMax=[]  NParamMin=[]  NParamMax=[]  KbParamMin=[]  KbParamMax=[]  KtParamMin=[]  KtParamMax=[]  KbOutMin=[]  KbOutMax=[]  KtOutMin=[]  KtOutMax=[]  IntegratorOutMin=[]  IntegratorOutMax=[]  FilterOutMin=[]  FilterOutMax=[]  SumI1OutMin=[]  SumI1OutMax=[]  SumI2OutMin=[]  SumI2OutMax=[]  SumI3OutMin=[]  SumI3OutMax=[]  SumI4OutMin=[]  SumI4OutMax=[]  SumDOutMin=[]  SumDOutMax=[]  DifferentiatorOutMin=[]  DifferentiatorOutMax=[]  FilterDiffOutCoefMin=[]  FilterDiffOutCoefMax=[]  ReciprocalOutMin=[]  ReciprocalOutMax=[]  SumDenOutMin=[]  SumDenOutMax=[]  SumNumOutMin=[]  SumNumOutMax=[]  DivideOutMin=[]  DivideOutMax=[]  UdiffTsProdOutMin=[]  UdiffTsProdOutMax=[]  NTsProdOutMin=[]  NTsProdOutMax=[]  UintegralTsProdOutMin=[]  UintegralTsProdOutMax=[]  UngainTsProdOutMin=[]  UngainTsProdOutMax=[]  ClampingZeroOutDataTypeStr=Inherit: Inherit via back propagation  ClampingZeroOutMin=[]  ClampingZeroOutMax=[]  FilterDenConstantOutDataTypeStr=Inherit: Inherit via back propagation  FilterDenConstantOutMin=[]  FilterDenConstantOutMax=[]  PCopyOutDataTypeStr=Inherit: Inherit via back propagation  PCopyOutMin=[]  PCopyOutMax=[]  NCopyOutDataTypeStr=Inherit: Inherit via back propagation  NCopyOutMin=[]  NCopyOutMax=[]  IntegratorContinuousStateAttributes=''  IntegratorStateMustResolveToSignalObject=off  IntegratorRTWStateStorageClass=Auto  FilterContinuousStateAttributes=''  FilterStateMustResolveToSignalObject=off  FilterRTWStateStorageClass=Auto  ParallelPVariant=ExternalParameters  IdealPVariant=Disabled  IVariant=ExternalParameters  DVariant=Disabled  IntegratorVariant=Discrete  SatVariant=Enabled  AWVariant=DiscClampingParallel  PCopyVariant=Disabled  TRVariant=Disabled  FdbkBlocksVariant=Forward  IdealPFdbkVariant=Disabled  SatFdbkVariant=Disabled  DerivativeFilterVariant=Disabled  NVariant=Disabled  NCopyVariant=Disabled_SignalSpec  FilterICVariant=Disabled  IntegratorICVariant=ExternalICs  ExternalResetVariant=ExternalReset  TRSumVariant=Passthrough  SumFdbkVariant=Disabled  SumVariant=Sum_PI  TsampFilterVariant=InternalTs  TsampNgainVariant=Passthrough  TsampIntegralVariant=Disabled_SignalSpec  ExternalSaturationOutDataTypeStr=Inherit: Same as second input
      settings: LibrarySourceBlock=mcbcontrolslib/PI Controller
  Ki : Constant  Commented=on  Value=PI_params.Ki_id*Ts  OutDataTypeStr=single  SampleTime=-1
  Ki1 : Constant  Commented=on  Value=0  OutDataTypeStr=single  SampleTime=-1
  Kp : Constant  Commented=on  Value=PI_params.Kp_id  OutDataTypeStr=single  SampleTime=-1
  Logical Operator : Logic  Commented=on  Operator=NOT  IconShape=distinctive  AllPortsSameDT=off  OutDataTypeStr=boolean
  PID Controller : slpidlib/PID Controller  Controller=PI  Form=Parallel  TimeDomain=Discrete-time  UseExternalTs=off  SampleTime=-1  IntegratorMethod=Forward Euler  FilterMethod=Forward Euler  ControllerParametersSource=internal  P=focp_tune_cur_Kp  I=focp_tune_cur_Ki  UseKiTs=off  D=0  N=100  UseFilter=on  TunerSelectOption=Transfer Function Based (PID Tuner App)  InitialConditionSource=internal  InitialConditionForIntegrator=0  InitialConditionForFilter=0  DifferentiatorICPrevScaledInput=0  ExternalReset=level  TrackingMode=off  Kt=1  LimitOutput=on  SatLimitsSource=internal  UpperSaturationLimit=1  LowerSaturationLimit=-1  LinearizeAsGain=off  AntiWindupMode=clamping  Kb=1  LimitIntegrator=off  UpperIntegratorSaturationLimit=inf  LowerIntegratorSaturationLimit=-inf  POutMin=[]  POutMax=[]  IOutMin=[]  IOutMax=[]  DOutMin=[]  DOutMax=[]  NOutMin=[]  NOutMax=[]  SumOutMin=[]  SumOutMax=[]  SaturationOutMin=[]  SaturationOutMax=[]  PParamDataTypeStr=fixdt(1,32,24)  PParamMin=[]  PParamMax=[]  IParamDataTypeStr=fixdt(1,32,16)  IParamMin=[]  IParamMax=[]  DParamMin=[]  DParamMax=[]  NParamMin=[]  NParamMax=[]  KbParamMin=[]  KbParamMax=[]  KtParamMin=[]  KtParamMax=[]  KbOutMin=[]  KbOutMax=[]  KtOutMin=[]  KtOutMax=[]  IntegratorOutMin=[]  IntegratorOutMax=[]  FilterOutMin=[]  FilterOutMax=[]  SumI1OutMin=[]  SumI1OutMax=[]  SumI2OutMin=[]  SumI2OutMax=[]  SumI3OutMin=[]  SumI3OutMax=[]  SumI4OutMin=[]  SumI4OutMax=[]  SumDOutMin=[]  SumDOutMax=[]  DifferentiatorOutMin=[]  DifferentiatorOutMax=[]  FilterDiffOutCoefMin=[]  FilterDiffOutCoefMax=[]  ReciprocalOutMin=[]  ReciprocalOutMax=[]  SumDenOutMin=[]  SumDenOutMax=[]  SumNumOutMin=[]  SumNumOutMax=[]  DivideOutMin=[]  DivideOutMax=[]  UdiffTsProdOutMin=[]  UdiffTsProdOutMax=[]  NTsProdOutMin=[]  NTsProdOutMax=[]  UintegralTsProdOutMin=[]  UintegralTsProdOutMax=[]  UngainTsProdOutMin=[]  UngainTsProdOutMax=[]  ClampingZeroOutDataTypeStr=Inherit: Inherit via back propagation  ClampingZeroOutMin=[]  ClampingZeroOutMax=[]  FilterDenConstantOutDataTypeStr=Inherit: Inherit via back propagation  FilterDenConstantOutMin=[]  FilterDenConstantOutMax=[]  PCopyOutDataTypeStr=Inherit: Inherit via back propagation  PCopyOutMin=[]  PCopyOutMax=[]  NCopyOutDataTypeStr=Inherit: Inherit via back propagation  NCopyOutMin=[]  NCopyOutMax=[]  IntegratorContinuousStateAttributes=''  IntegratorStateMustResolveToSignalObject=off  IntegratorRTWStateStorageClass=Auto  FilterContinuousStateAttributes=''  FilterStateMustResolveToSignalObject=off  FilterRTWStateStorageClass=Auto  ParallelPVariant=InternalParameters  IdealPVariant=Disabled  IVariant=InternalParameters  DVariant=Disabled  IntegratorVariant=Discrete  SatVariant=Enabled  AWVariant=DiscClampingParallel  PCopyVariant=Disabled  TRVariant=Disabled  FdbkBlocksVariant=Forward  IdealPFdbkVariant=Disabled  SatFdbkVariant=Disabled  DerivativeFilterVariant=Disabled  NVariant=Disabled  NCopyVariant=Disabled_SignalSpec  FilterICVariant=Disabled  IntegratorICVariant=InternalICs  ExternalResetVariant=ExternalReset  TRSumVariant=Passthrough  SumFdbkVariant=Disabled  SumVariant=Sum_PI  TsampFilterVariant=InternalTs  TsampNgainVariant=Passthrough  TsampIntegralVariant=Disabled_SignalSpec  ExternalSaturationOutDataTypeStr=Inherit: Same as second input
  Reset_I_Cur_And : Logic  AllPortsSameDT=off  OutDataTypeStr=boolean
  Reset_I_Cur_Enable : Constant  Value=ctrl_limits.reset_I_cur_freemode  OutDataTypeStr=boolean
  V_ref : Outport  VectorParamsAs1DForOutWhenUnconnected=off
  wires:
  Id_in/1 -> PID Controller/1
  PID Controller/1 -> V_ref/1
  Ki1/1 -> Discrete PI Controller with anti-windup & reset/5
  Logical Operator/1 -> Discrete PI Controller with anti-windup & reset/4
  Ki/1 -> Discrete PI Controller with anti-windup & reset/3
  Kp/1 -> Discrete PI Controller with anti-windup & reset/2
  Data Store Read1/1 -> Logical Operator/1
  [FreemodeSig_I] -> Reset_I_Cur_And/1
  Reset_I_Cur_Enable/1 -> Reset_I_Cur_And/2
  Reset_I_Cur_And/1 -> PID Controller/2
